simulink model "Zadanie_1_sim"  (R2026a)
settings: Solver=VariableStepAuto  StopTime=120
values from neighbouring files (symbols this model uses):
  A = [      -Ra/La,  -Kb/La,   0 ... (first row only)    [Zadanie_1.m]
  B = [      1/La ... (first row only)    [Zadanie_1.m]
  den = [      La*Jm,      Ra*Jm + La*Bm,      Ra*Bm + Kt*Kb,      0  ]    [Zadanie_1.m]
  Gde = 0.8    [Zadanie_1.m]
  Ge = 1/Ref    (= 0.381971863421)    [Zadanie_1.m]
  GKi = 20    [Zadanie_1.m]
  GKp = 130    [Zadanie_1.m]
  K_lqr = lqr(A, B, Q, R)    [Zadanie_1.m]
  Kd = C_pid.Kd    [Zadanie_1.m]
  Ki = C_pid.Ki    [Zadanie_1.m]
  Kp = C_pid.Kp    [Zadanie_1.m]
  num = Kt    (= 138)    [Zadanie_1.m]
  Ref = Deg*pi/180    (= 2.61799387799)    [Zadanie_1.m]
libraries: fuzblock x1, slpidlib x1
settings Model: Creator=Administrator  LastModifiedBy=Administrator

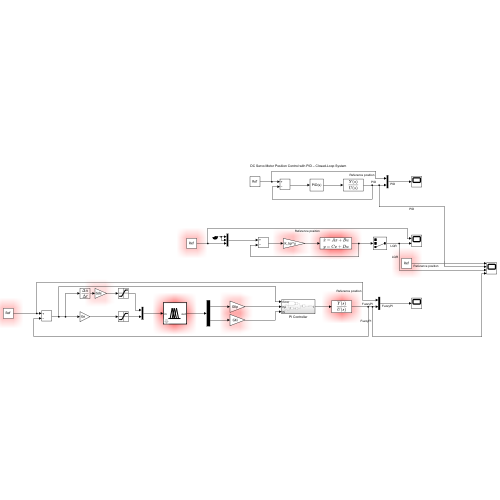
[thumbnail: Simulink's stored preview of the top-level diagram]
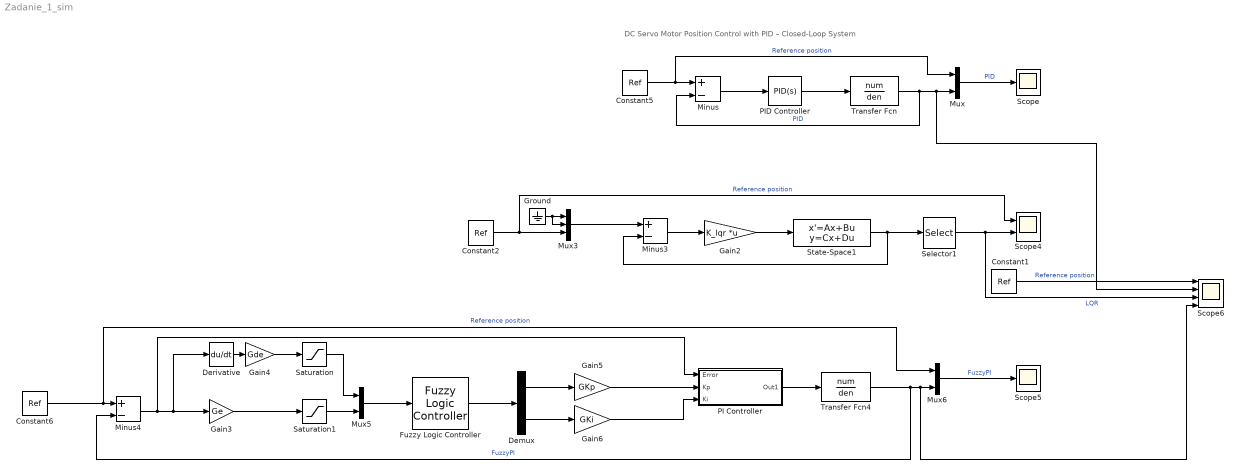
== system Zadanie_1_sim ==
  note: DC Servo Motor Position Control with PID – Closed-Loop System
  Constant{1..2,5..6} (4 alike) : Constant  Value=Ref
  Demux : Demux  Outputs=2
  Derivative : Derivative
  Fuzzy Logic Controller : fuzblock/Fuzzy Logic  Controller  FIS=Fuzzy_PI  OutputSampleNumber=101  DataType=double  UseLookupTable=off  NumBreakpoints=10  FuzzifiedInputs=off  RuleFiringStrengths=off  RuleOutputs=off  AggregatedOutputs=off  SimulateUsing=Interpreted execution  OutOfRangeInputValueMessage=warning  NoRuleFiredMessage=warning  EmptyOutputFuzzySetMessage=warning
  Gain2 : Gain  Gain=K_lqr  Multiplication=Matrix(K*u)
  Gain3 : Gain  Gain=Ge
  Gain4 : Gain  Gain=Gde
  Gain5 : Gain  Gain=GKp
  Gain6 : Gain  Gain=GKi
  Ground : Ground
  Minus : Sum  Inputs=+-
  Minus3 : Sum  Inputs=+-
  Minus4 : Sum  Inputs=+-
  Mux : Mux  Inputs=2
  Mux3 : Mux  Inputs=3
  Mux5 : Mux  Inputs=2
  Mux6 : Mux  Inputs=2
  PI Controller : Subsystem
  PID Controller : slpidlib/PID Controller  Controller=PID  Form=Parallel  TimeDomain=Continuous-time  UseExternalTs=off  SampleTime=-1  IntegratorMethod=Forward Euler  FilterMethod=Forward Euler  ControllerParametersSource=internal  P=Kp  I=Ki  UseKiTs=off  D=Kd  UseExternalDerivativeSource=off  N=100  UseFilter=on  TunerSelectOption=Transfer Function Based (PID Tuner App)  InitialConditionSource=internal  InitialConditionForIntegrator=0  InitialConditionForFilter=0  DifferentiatorICPrevScaledInput=0  ExternalReset=none  TrackingMode=off  Kt=1  LimitOutput=off  SatLimitsSource=internal  UpperSaturationLimit=inf  LowerSaturationLimit=-inf  LinearizeAsGain=on  AntiWindupMode=none  Kb=1  LimitIntegrator=off  UpperIntegratorSaturationLimit=inf  LowerIntegratorSaturationLimit=-inf  POutMin=[]  POutMax=[]  IOutMin=[]  IOutMax=[]  DOutMin=[]  DOutMax=[]  NOutMin=[]  NOutMax=[]  SumOutMin=[]  SumOutMax=[]  SaturationOutMin=[]  SaturationOutMax=[]  PParamMin=[]  PParamMax=[]  IParamMin=[]  IParamMax=[]  DParamMin=[]  DParamMax=[]  NParamMin=[]  NParamMax=[]  KbParamMin=[]  KbParamMax=[]  KtParamMin=[]  KtParamMax=[]  KbOutMin=[]  KbOutMax=[]  KtOutMin=[]  KtOutMax=[]  IntegratorOutMin=[]  IntegratorOutMax=[]  FilterOutMin=[]  FilterOutMax=[]  SumI1OutMin=[]  SumI1OutMax=[]  SumI2OutMin=[]  SumI2OutMax=[]  SumI3OutMin=[]  SumI3OutMax=[]  SumI4OutMin=[]  SumI4OutMax=[]  SumDOutMin=[]  SumDOutMax=[]  DifferentiatorOutMin=[]  DifferentiatorOutMax=[]  FilterDiffOutCoefMin=[]  FilterDiffOutCoefMax=[]  ReciprocalOutMin=[]  ReciprocalOutMax=[]  SumDenOutMin=[]  SumDenOutMax=[]  SumNumOutMin=[]  SumNumOutMax=[]  DivideOutMin=[]  DivideOutMax=[]  UdiffTsProdOutMin=[]  UdiffTsProdOutMax=[]  NTsProdOutMin=[]  NTsProdOutMax=[]  UintegralTsProdOutMin=[]  UintegralTsProdOutMax=[]  UngainTsProdOutMin=[]  UngainTsProdOutMax=[]  ClampingZeroOutDataTypeStr=Inherit: Inherit via back propagation  ClampingZeroOutMin=[]  ClampingZeroOutMax=[]  FilterDenConstantOutDataTypeStr=Inherit: Inherit via back propagation  FilterDenConstantOutMin=[]  FilterDenConstantOutMax=[]  PCopyOutDataTypeStr=Inherit: Inherit via back propagation  PCopyOutMin=[]  PCopyOutMax=[]  NCopyOutDataTypeStr=Inherit: Inherit via back propagation  NCopyOutMin=[]  NCopyOutMax=[]  IntegratorContinuousStateAttributes=''  IntegratorStateMustResolveToSignalObject=off  IntegratorRTWStateStorageClass=Auto  FilterContinuousStateAttributes=''  FilterStateMustResolveToSignalObject=off  FilterRTWStateStorageClass=Auto  ParallelPVariant=InternalParameters  IdealPVariant=Disabled  IVariant=InternalParameters  DVariant=InternalParameters  IntegratorVariant=Continuous  SatVariant=Disabled  AWVariant=Passthrough  PCopyVariant=Disabled  TRVariant=Disabled  FdbkBlocksVariant=Forward  IdealPFdbkVariant=Disabled  SatFdbkVariant=Disabled  DerivativeFilterVariant=ContFilter  NVariant=InternalParameters  NCopyVariant=Disabled  FilterICVariant=InternalICsFilter  IntegratorICVariant=InternalICs  ExternalResetVariant=Disabled  TRSumVariant=Passthrough  SumFdbkVariant=Disabled  SumVariant=Sum_PID  TsampFilterVariant=InternalTs  TsampNgainVariant=Passthrough  TsampIntegralVariant=Disabled_SignalSpec  ExternalSaturationOutDataTypeStr=Inherit: Same as second input  DerivativeSourceVariant=ErrorSignal  PreIntVariant=InternalPreInt
  Saturation : Saturate  UpperLimit=1  LowerLimit=-1
  Saturation1 : Saturate  UpperLimit=1  LowerLimit=-1
  Scope : Scope
      settings: ActiveDisplayYMinimum=-0.41707599004262358  ActiveDisplayYMaximum=3.753683910383613
  Scope4 : Scope  NumInputPorts=2
      settings: ActiveDisplayYMinimum=-0.54835051429747361  ActiveDisplayYMaximum=2.9698099215791576  DataLoggingVariableName=ScopeData4
  Scope5 : Scope
      settings: ActiveDisplayYMinimum=-0.482571611076611  ActiveDisplayYMaximum=4.3431444996895  DataLoggingVariableName=ScopeData5
  Scope6 : Scope  NumInputPorts=4
      settings: ActiveDisplayYMinimum=-0.41750975741478  ActiveDisplayYMaximum=3.7575878167330212  DataLoggingVariableName=ScopeData6
  Selector1 : Selector  InputPortWidth=3  IndexOptions=Index vector (dialog)  Indices=3  OutputSizes=1
  State-Space1 : StateSpace  A=A  B=B  C=eye(3)  D=zeros(3,1)  InitialCondition=0
  Transfer Fcn : TransferFcn  Numerator=num  Denominator=den
  Transfer Fcn4 : TransferFcn  Numerator=num  Denominator=den
  wires:
  Constant5/1 -> Mux/1, Minus/1  "Reference position"
  Minus/1 -> PID Controller/1
  PID Controller/1 -> Transfer Fcn/1
  Transfer Fcn/1 -> Scope6/2, Mux/2, Minus/2  "PID"
  Mux/1 -> Scope/1  "PID"
  Constant2/1 -> Scope4/1, Mux3/3  "Reference position"
  Mux3/1 -> Minus3/1
  Minus3/1 -> Gain2/1
  Gain2/1 -> State-Space1/1
  State-Space1/1 -> Selector1/1, Minus3/2
  Ground/1 -> Mux3/2, Mux3/1
  Constant6/1 -> Mux6/1, Minus4/1  "Reference position"
  Minus4/1 -> PI Controller/1(Error), Derivative/1, Gain3/1
  Derivative/1 -> Gain4/1
  Mux5/1 -> Fuzzy Logic Controller/1
  Fuzzy Logic Controller/1 -> Demux/1
  Demux/1 -> Gain5/1
  Demux/2 -> Gain6/1
  Transfer Fcn4/1 -> Scope6/4, Mux6/2, Minus4/2  "FuzzyPI"
  Mux6/1 -> Scope5/1  "FuzzyPI"
  Gain5/1 -> PI Controller/2(Kp)
  Gain6/1 -> PI Controller/3(Ki)
  PI Controller/1(Out1) -> Transfer Fcn4/1
  Gain4/1 -> Saturation/1
  Saturation/1 -> Mux5/1
  Gain3/1 -> Saturation1/1
  Saturation1/1 -> Mux5/2
  Selector1/1 -> Scope6/3, Scope4/2  "LQR"
  Constant1/1 -> Scope6/1  "Reference position"

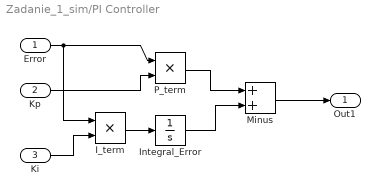
== system Zadanie_1_sim/PI Controller ==
  Error : Inport
  Kp : Inport  Port=2
  Ki : Inport  Port=3
  I_term : Product
  Integral_Error : Integrator
  Minus : Sum
  P_term : Product
  Out1 : Outport
  wires:
  Error/1 -> I_term/1, P_term/1
  Kp/1 -> P_term/2
  Ki/1 -> I_term/2
  P_term/1 -> Minus/1
  Minus/1 -> Out1/1
  I_term/1 -> Integral_Error/1
  Integral_Error/1 -> Minus/2
